simulink model "testrig_quarter_car"  (R2025b)
settings: Solver=ode23t  StartTime=0.0  StopTime=96  MaxStep=0.1  RelTol=1e-3  AbsTol=1e-3  EnableMultiTasking=on
PostLoadFcn:
  | Maneuver = MDatabase.KnC.FSAE_Achilles;
values from neighbouring files (symbols this model uses):
  Vehicle = evalin('base','Vehicle')    [sm_car_knc_plot1toecamber.m]    (also in testrig_quarter_car_results.m = sm_car_vehcfg_setPeopleOnOff(Vehicle,[0 0 0 0 0],'SuspA1'))
undefined symbols (not defined in the file or in its folder): X, Y, Z
libraries: sm_lib x9, nesl_utility x6, fl_lib x6, sm_car_testrig_utilities_lib x5, Damper_Element x1, Linkage_Systems x1, Suspension_Utilities x1
CloseFcn:
  | clear simlog_sm_car_testrig_quarter_car
  | clear logsout_sm_car_testrig_quarter_car
  | evalin('base','Maneuver = MDatabase.Skidpad.FSAE_Achilles;')
Description:
  | Copyright 2020-2024 The MathWorks, Inc.
settings Model: Creator=smiller  LastModifiedBy=andrei
settings SolverCC: AutoScaleAbsTol=off  AlgebraicLoopSolver=TrustRegion
settings DataIOCC: LimitDataPoints=on  MaxDataPoints=10000  ReturnWorkspaceOutputs=off  SignalLoggingName=logsout_sm_car_testrig_quarter_car
settings OptimizationCC: LifeSpan=inf
settings DebuggingCC: UnconnectedInputMsg=warning  UnconnectedOutputMsg=warning  UnconnectedLineMsg=warning  AllowSymbolicDim=off  SFUnexpectedBacktrackingDiag=warning  SFNoUnconditionalDefaultTransitionDiag=warning  SFExecutionAtInitializationDiag=none  ArithmeticOperatorsInVariantConditions=warning
settings ModelReferenceCC: EnableRefExpFcnMdlSchedulingChecks=on
settings SFSimCC: SimUseLocalCustomCode=off  CustomCodeUndefinedFunction=UseInterfaceOnly
settings RTWCC: RTWUseLocalCustomCode=off  GPUComputeCapability=3.5
settings CodeAppCC: StateflowObjectComments=on
settings GRTTargetCC: TargetLangStandard=C89/C90 (ANSI)
settings ConfigComp: CovMetricSettings=dw  CovSaveCumulativeToWorkspaceVar=on  CovSaveSingleToWorkspaceVar=on  CovExternalEMLEnable=off  CovSFcnEnable=off
settings SimscapeCC: SimscapeLogType=all  SimscapeLogSimulationStatistics=on  SimscapeLogName=simlog_sm_car_testrig_quarter_car  SimscapeLogDataHistory=10000.0
settings DiagnosticsConfigSet: SimMechanicsUnconnectedFramePorts=none
settings ExplorerConfigSet: InternalSimMechanicsExplorerSettings="<ExplorerConfiguration><canonicalview>default</canonicalview><AnimationSetting><BasePlaybackSpeed>1.0</BasePlaybackSpeed><PlaybackSpeedFactor>16.0</PlaybackSpeedFactor></AnimationSetting><TilePanel><TileInfo><Tiles Columns=\"1\" Count=\"1\" Rows=\"1\"><Column Weight=\"1\"/><Row Weight=\"1\"/><Tile Height=\"1\" Width=\"1\" X=\"0\" Y=\"0\"/></Tiles></TileInfo><SceneInfo><SceneViewer><BGColor><R>1</R><G>1</G><B>1</B></BGColor><Camera><DoPerspective>off</DoPerspective><Position><X>-1.00754384696483612</X><Y>0.620980322360992432</Y><Z>0.415903732180595842</Z></Position><Center><X>-0.00754384696483612061</X><Y>0.620980322360992432</Y><Z>0.415903732180595842</Z></Center><Up><X>0</X><Y>0</Y><Z>1</Z></Up><ViewLimDist>1</ViewLimDist><YLim>0.446366462798987951</YLim><XLim>0.523904299059845036</XLim></Camera></SceneViewer></SceneInfo></TilePanel><MechEditorPanel><Cameras/><GfxPanelCameraMap/><VideoCreator><PlaybackSpeedRatio>1.0</PlaybackSpeedRatio><FrameRate>30</FrameRate><VideoFormat>Motion JPEG AVI</VideoFormat><FrameSize>auto</FrameSize></VideoCreator></MechEditorPanel></ExplorerConfiguration>"

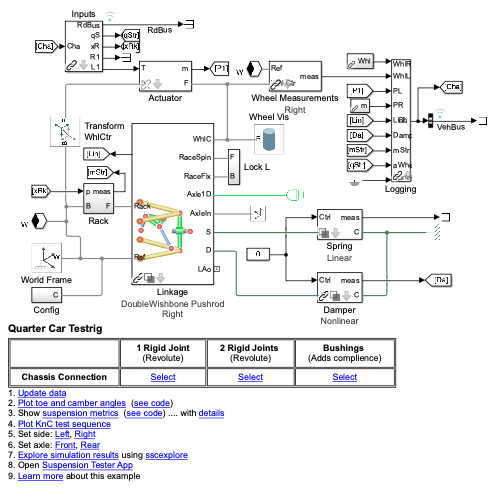
[thumbnail: Simulink's stored preview of the top-level diagram]
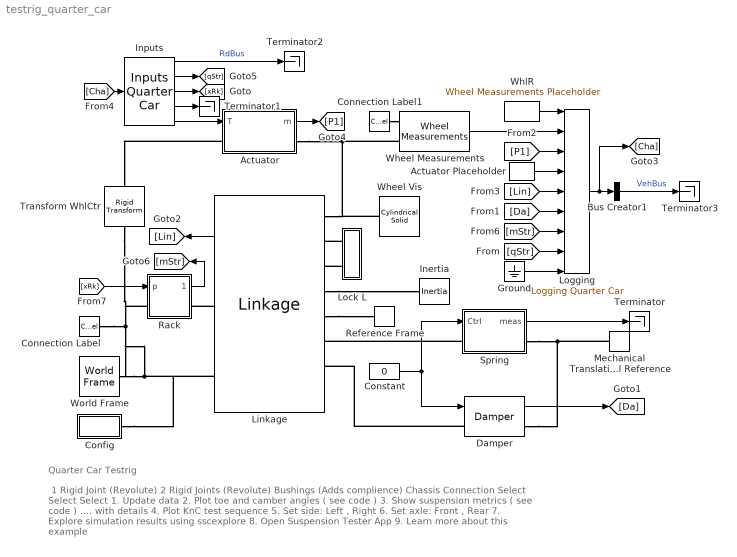
== system testrig_quarter_car ==
  note: Quarter Car Testrig
  note: ​
      | 1 Rigid Joint
      | (Revolute)
      | 2 Rigid Joints
      | (Revolute)
      | Bushings
      | (Adds complience)
      |
      | Chassis Connection
      | Select
      | Select
      | Select
      |
      | 1. Update data
      | 2. Plot toe and camber angles ( see code )
      | 3. Show suspension metrics ( see code ) .... with details
      | 4. Plot KnC test sequence
      | 5. Set side: Left , Right
      | 6. Set axle: Front , Rear
      | 7. Explore simulation results using sscexplore
      | 8. Open Suspension Tester App
      | 9. Learn more about this example
  Actuator : Subsystem  AncestorBlock=sm_car_testrig_utilities_lib/Actuator Quarter Car  mask{veh=Vehicle, xCPOffset=Maneuver.xCPOffset, tir_file=Vehicle.Chassis.Tire.tirFile.Value}
      mask prompts: veh "Vehicle (structure)"; xCPOffset "xOffset from Contact Patch for force test (m)"; tir_file "Tire File"
      mask init:
      | tire_param = simscape.multibody.tirread(eval(tir_file));
      | tire_radius = tire_param.DIMENSION.UNLOADED_RADIUS;
      mask TypeOptions xCPOffset: Actuator/xCPOffset
  Actuator Placeholder : sm_car_testrig_utilities_lib/Actuator Placeholder  SystemSampleTime=-1  VariantActivationTime=update diagram  EmptyChoice=off  PassThrough=off  PassThroughVariantControl=(default)  EmptyChoiceVariantControl=(default)  AllowFlexibleInterface=on  Latency=0  AutoFrameSizeCalculation=off
  Bus Creator1 : BusCreator  Inputs=1
  Config : Subsystem
  Connection Label : ConnectionLabel  Label=W
  Connection Label1 : ConnectionLabel  Label=W
  Constant : Constant  Value=0
  Damper : Damper_Element/Damper  VariantControl=Variant1  LabelModeActiveChoice=Nonlinear  Damper=Vehicle.Chassis.Damper.Axle1  VariantLabel=Vehicle.Chassis.Damper.Axle1.class.Value
      settings: AttributesFormatString=%<ActiveVariant>
  Ground : Ground
  Inertia : fl_lib/Mechanical/Rotational Elements/Inertia  inertia=0.01 kg*m^2  num_ports=foundation.enum.numPorts2.one  w_specify=on  w_priority=None  w=0 rad/s  w_nominal_specify=off  w_nominal_value=1  w_nominal_unit=rad/s  t_specify=off  t_priority=None  t=0 N*m  t_nominal_specify=off  t_nominal_value=1  t_nominal_unit=N*m
  Inputs : sm_car_testrig_utilities_lib/Inputs Quarter Car  popup_steering_input=On
  Linkage : Linkage_Systems/Linkage  VariantControl=Variant1  LabelModeActiveChoice=DoubleWishbone Pushrod  popup_leftRight=Right  Linkage=Vehicle.Chassis.SuspA1.Linkage  InitLinkage=Init.Axle1  VariantLabel=Vehicle.Chassis.SuspA1.Linkage.class.Value
      settings: AttributesFormatString=|
      | %<ActiveVariant>
      | %<popup_leftRight>
  Lock L : Subsystem
  Logging : sm_car_testrig_utilities_lib/Logging Quarter Car
  Mechanical Translational Reference : fl_lib/Mechanical/Translational Elements/Mechanical Translational Reference
  Rack : Subsystem
  Reference Frame : sm_lib/Frames and Transforms/Reference Frame
  Spring : Subsystem  Variant=on  VariantControlMode=label  VariantControl=Variant1  LabelModeActiveChoice=Linear  mask(Variants for Spring){Spring=Vehicle.Chassis.Spring.Axle1, VariantLabel=Vehicle.Chassis.Spring.Axle1.class.Value}
      mask prompts: Spring "Spring Parameters"; VariantLabel "Variant Label"
      mask help: Select option and provide parameters for spring. Option is chosen by string provided in Variant Label. The parameters for the selected option is contained in Spring data structure.
      mask init:
      | curblk = gcb;
      | 
      | % Set variant for this block 
      | set_param(curblk,'LabelModeActiveChoice',VariantLabel);
      settings: AttributesFormatString=%<ActiveVariant>
      mask Display: disp(' ')
  Terminator{,1..3} (4 alike) : Terminator
  Transform WhlCtr : sm_lib/Frames and Transforms/Rigid Transform  RotationMethod=None  FollAlignAxisA=+X  BaseAlignAxisA=+Y  FollAlignAxisB=+Y  BaseAlignAxisB=+Z  RotationStandardAxis=+Z  RotationAngle=0.0  RotationAngleUnits=deg  RotationArbitraryAxis=[0 0 1]  RotationSequenceAxes=FollowerAxes  RotationSequence=XYX  RotationSequenceAngles=[0 0 0]  RotationSequenceAnglesUnits=deg  RotationMatrix=[1 0 0; 0 1 0; 0 0 1]  Quaternion=[1 0 0 0]  TranslationMethod=StandardAxis  TranslationCartesianOffset=[0 0 0]  TranslationCartesianOffsetUnits=m  TranslationStandardAxis=+Z  TranslationStandardOffset=Vehicle.Chassis.SuspA1.Linkage.Upright.sWheelCentre.Value(3)  TranslationStandardOffsetUnits=m  TranslationROffset=0  TranslationROffsetUnits=m  TranslationThetaOffset=0  TranslationThetaOffsetUnits=deg  TranslationZOffset=0  TranslationZOffsetUnits=m
  Wheel Measurements : Suspension_Utilities/Wheel Measurements  popup_leftRight=Right
      settings: AttributesFormatString=%<popup_leftRight>  SourceProductName=SmCar - Suspension Utilites
  Wheel Vis : sm_lib/Body Elements/Cylindrical Solid  CylinderRadius=0.23  CylinderRadiusUnits=m  CylinderLength=0.25  CylinderLengthUnits=m  ExportEntireGeometry=off  InertiaType=CalculateFromGeometry  BasedOnType=Mass  Density=1000  DensityUnits=kg/m^3  Mass=10  MassUnits=kg  CenterOfMass=[0 0 0]  CenterOfMassUnits=m  MomentsOfInertia=[1 1 1]  MomentsOfInertiaUnits=kg*m^2  ProductsOfInertia=[0 0 0]  ProductsOfInertiaUnits=kg*m^2  GraphicType=FromGeometry  MarkerShape=Sphere  MarkerSize=10  GraphicVisPropType=SimpleVisualProperties  GraphicDiffuseColor=[0.5 0.5 0.5]  GraphicOpacity=0.3  GraphicSpecularColor=[0.5 0.5 0.5 1.0]  GraphicAmbientColor=[0.15 0.15 0.15 1.0]  GraphicEmissiveColor=[0.0 0.0 0.0 1.0]  GraphicShininess=75  DoExposeReferenceFrame=on  SerializedFrames=<Frames/>
  WhlR : sm_car_testrig_utilities_lib/Wheel Measurements Placeholder  SystemSampleTime=-1  VariantActivationTime=update diagram  EmptyChoice=off  PassThrough=off  PassThroughVariantControl=(default)  EmptyChoiceVariantControl=(default)  AllowFlexibleInterface=on  Latency=0  AutoFrameSizeCalculation=off
  World Frame : sm_lib/Frames and Transforms/World Frame
  wires:
  Constant/1 -> Spring/1("Ctrl "), Damper/1
  Spring/1(" meas") -> Terminator/1
  Linkage/1 -> [Lin]
  Bus Creator1/1 -> Terminator3/1  "VehBus"
  [xRk] -> Rack/1(p)
  Damper/1 -> [Da]
  Wheel Measurements/1 -> Logging/2
  Inputs/1 -> Terminator2/1  "RdBus"
  Inputs/3 -> [xRk]
  Inputs/4 -> Terminator1/1
  [Cha] -> Inputs/1
  Inputs/2 -> [qStr]
  Logging/1 -> [Cha], Bus Creator1/1
  [qStr] -> Logging/8
  [mStr] -> Logging/7
  [Da] -> Logging/6
  [Lin] -> Logging/5
  [P1] -> Logging/3
  WhlR/1 -> Logging/1
  Ground/1 -> Logging/9
  Actuator Placeholder/1 -> Logging/4
  Rack/1(meas) -> [mStr]
  Inputs/5 -> Actuator/1(T)
  Actuator/1(m) -> [P1]
  connections:
  Wheel Vis/RConn1 -- Linkage/LConn1 -- Actuator/RConn1 -- Wheel Measurements/LConn2
  Mechanical Translational Reference/LConn1 -- Spring/RConn1 -- Damper/RConn1
  World Frame/RConn1 -- Linkage/RConn2 -- Config/RConn1 -- Rack/LConn1 -- Transform WhlCtr/LConn1 -- Connection Label/LConn1
  Spring/LConn1 -- Linkage/LConn6
  Linkage/LConn4 -- Inertia/LConn1
  Linkage/LConn5 -- Reference Frame/RConn1
  Damper/LConn1 -- Linkage/LConn7
  Linkage/RConn1 -- Rack/RConn1
  Lock L/LConn1 -- Linkage/LConn2
  Lock L/LConn2 -- Linkage/LConn3
  Connection Label1/LConn1 -- Wheel Measurements/LConn1
  Actuator/LConn1 -- Transform WhlCtr/RConn1

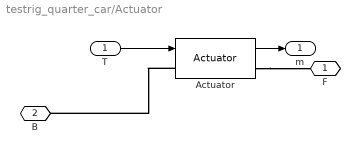
== system testrig_quarter_car/Actuator ==
  T : Inport
  Actuator : sm_car_testrig_utilities_lib/Actuator  tire_rad=tire_radius  xCPOffset=xCPOffset
  F : PMIOPort  Side=Right
  B : PMIOPort  Port=2  Side=Left
  m : Outport
  wires:
  T/1 -> Actuator/1
  Actuator/1 -> m/1
  connections:
  Actuator/RConn1 -- F/RConn1
  Actuator/LConn1 -- B/RConn1

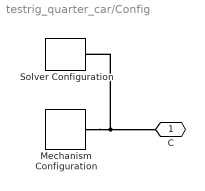
== system testrig_quarter_car/Config ==
  Mechanism Configuration : sm_lib/Utilities/Mechanism Configuration  UniformGravity=Constant  GravityVector=[0 0 -9.80665]  GravityVectorUnits=m/s^2  LinearizationDelta=0.001  JointModeTransitionNonlinearIterations=2
  Solver Configuration : nesl_utility/Solver Configuration  PhysicalDomain=network_engine_domain  SubClassName=solver  LeftPortType=input  RightPortType=generic  Tones=[]  Harmonics=[]  SimulateNoise=off  Profile=off  UseLocalSampling=off  EnableSwitchedLinearOptims=on  FrequencyDomain=off  UseCCode=off  RelTol=0.001  AbsTol=1e-06  MinStep=1e-09  ToWorkspace=off  RevertToSquareIcSolve=off  NumHomotopyIterations=100  PhasorMode=off  PhasorModeNumHarmonics=1  ConsistencySolver=NEWTON_FTOL  IndexReductionMethod=DerivativeReplacement  DoDC=off  ResidualTolerance=1e-09  ConsistencyTolSource=GLOBAL  ConsistencyAbsTol=0.001  ConsistencyRelTol=0.001  ConsistencyTolFactor=0.001  UseLocalSolver=off  LocalSolverChoice=NE_BACKWARD_EULER_ADVANCER  ResolveIndetEquations=on  FunctionEvalNumThread=1  LocalSolverSampleTime=0.001  DoFixedCost=off  MaxNonlinIter=3  MaxModeIter=2  ComputeImpulses=off  ImpulseIterations=2  LinearAlgebra=Sparse  LinearAlgebraNumThread=0  EquationFormulation=NE_TIME_EF  DelaysMemoryBudget=1024  AutomaticFiltering=on  FilteringTimeConstant=0.001  PartitionStorageMethod=AS_NEEDED  PartitionMemoryBudget=1024  PartitionMethod=FAST  MultibodyUseLocalSolver=off  MultibodyLocalSolverChoice=ODE1  MultibodyLocalSolverSampleTime=0.001
  C : PMIOPort  Side=Right
  connections:
  Mechanism Configuration/RConn1 -- Solver Configuration/RConn1 -- C/RConn1

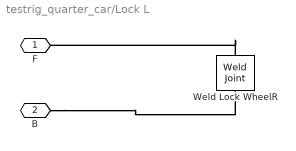
== system testrig_quarter_car/Lock L ==
  Weld Lock WheelR : sm_lib/Joints/Weld Joint  JointMode=Normal  CompositeWrenchDir=FollowerOnBase  CompositeWrenchFrame=BaseFrame  SenseConstraintForce=off  SenseConstraintTorque=off  SenseTotalForce=off  SenseTotalTorque=off
  F : PMIOPort  Side=Left
  B : PMIOPort  Port=2  Side=Left
  connections:
  B/RConn1 -- Weld Lock WheelR/LConn1
  Weld Lock WheelR/RConn1 -- F/RConn1

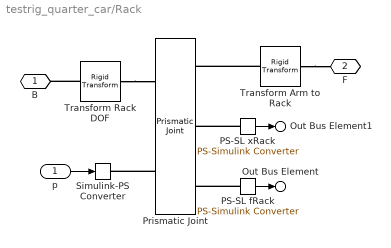
== system testrig_quarter_car/Rack ==
  p : Inport
  PS-SL fRack : nesl_utility/PS-Simulink Converter  PhysicalDomain=network_engine_domain  SubClassName=ps_output  LeftPortType=input  RightPortType=output  PseudoPeriodic=off  Frequencies=[]  VectorFormat=1-D array  Unit=1  AffineConversion=off
  PS-SL xRack : nesl_utility/PS-Simulink Converter  PhysicalDomain=network_engine_domain  SubClassName=ps_output  LeftPortType=input  RightPortType=output  PseudoPeriodic=off  Frequencies=[]  VectorFormat=1-D array  Unit=1  AffineConversion=off
  Prismatic Joint : sm_lib/Joints/Prismatic Joint  JointMode=Normal  CompositeWrenchDir=FollowerOnBase  CompositeWrenchFrame=BaseFrame  SenseConstraintForce=off  SenseConstraintTorque=off  SenseTotalForce=off  SenseTotalTorque=off  PositionTargetSpecify=on  PositionTargetPriority=High  PositionTargetValue=0  PositionTargetValueUnits=m  VelocityTargetSpecify=off  VelocityTargetPriority=High  VelocityTargetValue=0  VelocityTargetValueUnits=m/s  EquilibriumPosition=0  EquilibriumPositionUnits=m  SpringStiffness=0  SpringStiffnessUnits=N/m  DampingCoefficient=0  DampingCoefficientUnits=N/(m/s)  LowerLimitSpecify=off  LowerLimitBound=-1  LowerLimitBoundUnits=m  LowerLimitStiffness=1e6  LowerLimitStiffnessUnits=N/m  LowerLimitDamping=1e3  LowerLimitDampingUnits=N/(m/s)  LowerLimitTransitionRegionWidth=1e-4  LowerLimitTransitionRegionWidthUnits=m  UpperLimitSpecify=off  UpperLimitBound=1  UpperLimitBoundUnits=m  UpperLimitStiffness=1e6  UpperLimitStiffnessUnits=N/m  UpperLimitDamping=1e3  UpperLimitDampingUnits=N/(m/s)  UpperLimitTransitionRegionWidth=1e-4  UpperLimitTransitionRegionWidthUnits=m  TorqueActuationMode=ComputedTorque  MotionActuationMode=InputMotion  SensePosition=on  SenseVelocity=off  SenseAcceleration=off  SenseTorqueForce=on  SenseLowerLimitTorqueForce=off  SenseUpperLimitTorqueForce=off
  Simulink-PS Converter : nesl_utility/Simulink-PS Converter  PhysicalDomain=network_engine_domain  SubClassName=ps_input  LeftPortType=input  RightPortType=output  PseudoPeriodic=off  Frequencies=[]  NoiseDistribution=none  NoiseParameters=[]  Unit=m  AffineConversion=off  FilteringAndDerivatives=filter  SimscapeFilterOrder=2  InputFilterTimeConstant=0.005  UdotUserProvided=0
  Transform Arm to Rack : sm_lib/Frames and Transforms/Rigid Transform  RotationMethod=StandardAxis  FollAlignAxisA=+X  BaseAlignAxisA=+Y  FollAlignAxisB=+Y  BaseAlignAxisB=+Z  RotationStandardAxis=+X  RotationAngle=90  RotationAngleUnits=deg  RotationArbitraryAxis=[0 0 1]  RotationSequenceAxes=FollowerAxes  RotationSequence=XYX  RotationSequenceAngles=[0 0 0]  RotationSequenceAnglesUnits=deg  RotationMatrix=[1 0 0; 0 1 0; 0 0 1]  Quaternion=[1 0 0 0]  TranslationMethod=Cartesian  TranslationCartesianOffset=Vehicle.Chassis.SuspA1.Linkage.TrackRod.sInboard.Value.*[1 0 1]  TranslationCartesianOffsetUnits=m  TranslationStandardAxis=+Z  TranslationStandardOffset=0  TranslationStandardOffsetUnits=m  TranslationROffset=0  TranslationROffsetUnits=m  TranslationThetaOffset=0  TranslationThetaOffsetUnits=deg  TranslationZOffset=0  TranslationZOffsetUnits=m
  Transform Rack DOF : sm_lib/Frames and Transforms/Rigid Transform  RotationMethod=StandardAxis  FollAlignAxisA=+X  BaseAlignAxisA=+Y  FollAlignAxisB=+Y  BaseAlignAxisB=+Z  RotationStandardAxis=+X  RotationAngle=90  RotationAngleUnits=deg  RotationArbitraryAxis=[0 0 1]  RotationSequenceAxes=FollowerAxes  RotationSequence=XYX  RotationSequenceAngles=[0 0 0]  RotationSequenceAnglesUnits=deg  RotationMatrix=[1 0 0; 0 1 0; 0 0 1]  Quaternion=[1 0 0 0]  TranslationMethod=Cartesian  TranslationCartesianOffset=Vehicle.Chassis.SuspA1.Linkage.TrackRod.sInboard.Value.*[1 0 1]  TranslationCartesianOffsetUnits=m  TranslationStandardAxis=+Z  TranslationStandardOffset=0  TranslationStandardOffsetUnits=m  TranslationROffset=0  TranslationROffsetUnits=m  TranslationThetaOffset=0  TranslationThetaOffsetUnits=deg  TranslationZOffset=0  TranslationZOffsetUnits=m
  B : PMIOPort  Side=Left
  F : PMIOPort  Port=2  Side=Right
  Out Bus Element : Outport  VectorParamsAs1DForOutWhenUnconnected=off  PortName=meas  Element=FRack
  Out Bus Element1 : Outport  VectorParamsAs1DForOutWhenUnconnected=off  PortName=meas  Element=xRack
  wires:
  p/1 -> Simulink-PS Converter/1
  PS-SL fRack/1 -> Out Bus Element/1
  PS-SL xRack/1 -> Out Bus Element1/1
  connections:
  Transform Rack DOF/RConn1 -- Prismatic Joint/LConn1
  Prismatic Joint/LConn2 -- Simulink-PS Converter/RConn1
  Transform Arm to Rack/LConn1 -- F/RConn1
  Transform Arm to Rack/RConn1 -- Prismatic Joint/RConn1
  Transform Rack DOF/LConn1 -- B/RConn1
  PS-SL xRack/LConn1 -- Prismatic Joint/RConn2
  PS-SL fRack/LConn1 -- Prismatic Joint/RConn3

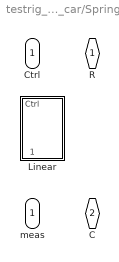
== system testrig_quarter_car/Spring ==
  "Ctrl " : Inport
  Linear : Subsystem  VariantControl=Linear  mask(Linear Spring){spr_def0=Spring.xPreload.Value, spr_k=Spring.K.Value, spr_hp_top=Spring.sTop.Value, spr_hp_bot=Spring.sBottom.Value}
      mask prompts: spr_def0 "Spring Preload (m)"; spr_k "Spring Rate (N/m)"; spr_hp_top "HP Top [xyz] (m)"; spr_hp_bot "HP Bottom [xyz] (m)"
      mask help: Spring with linear stiffness.
      mask init:
      | spr_len0 = norm(spr_hp_top-spr_hp_bot);
  " R" : PMIOPort  Side=Left
  " C" : PMIOPort  Port=2  Side=Right
  " meas" : Outport  VectorParamsAs1DForOutWhenUnconnected=off

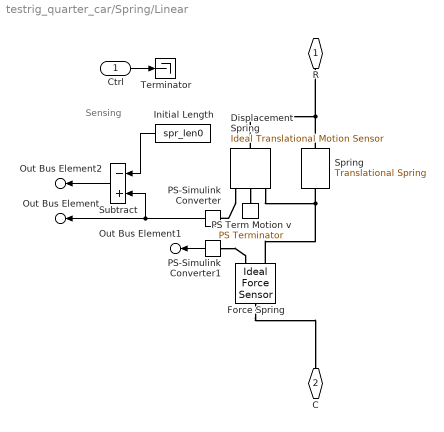
== system testrig_quarter_car/Spring/Linear ==
  note: Sensing
  Ctrl : Inport
  Displacement Spring : fl_lib/Mechanical/Mechanical Sensors/Ideal Translational Motion Sensor  reference=foundation.enum.MeasurementReference.difference  acceleration_port=false  velocity_port=true  position_port=true  offset=spr_len0 m
  Force Spring : fl_lib/Mechanical/Mechanical Sensors/Ideal Force Sensor
  Initial Length : Constant  Value=spr_len0
  PS Term Motion v : fl_lib/Physical Signals/Sinks/PS Terminator
  PS-Simulink Converter : nesl_utility/PS-Simulink Converter  PhysicalDomain=network_engine_domain  SubClassName=ps_output  LeftPortType=input  RightPortType=output  PseudoPeriodic=off  Frequencies=[]  VectorFormat=1-D array  Unit=m  AffineConversion=off
  PS-Simulink Converter1 : nesl_utility/PS-Simulink Converter  PhysicalDomain=network_engine_domain  SubClassName=ps_output  LeftPortType=input  RightPortType=output  PseudoPeriodic=off  Frequencies=[]  VectorFormat=1-D array  Unit=N  AffineConversion=off
  Spring : fl_lib/Mechanical/Translational Elements/Translational Spring  spr_rate=spr_k N/m  v_specify=off  v_priority=None  v=0 m/s  v_nominal_specify=off  v_nominal_value=1  v_nominal_unit=m/s  f_specify=off  f_priority=None  f=0 N  f_nominal_specify=off  f_nominal_value=1  f_nominal_unit=N  x_specify=on  x_priority=High  x=-spr_def0 m  x_nominal_specify=off  x_nominal_value=1  x_nominal_unit=m
  Subtract : Sum  Inputs=-+
  Terminator : Terminator
  R : PMIOPort  Side=Left
  C : PMIOPort  Port=2  Side=Right
  Out Bus Element : Outport  VectorParamsAs1DForOutWhenUnconnected=off  PortName=meas  Element=xSpring
  Out Bus Element1 : Outport  VectorParamsAs1DForOutWhenUnconnected=off  PortName=meas  Element=FSpring
  Out Bus Element2 : Outport  VectorParamsAs1DForOutWhenUnconnected=off  PortName=meas  Element=DeltaxSpring
  wires:
  PS-Simulink Converter/1 -> Out Bus Element/1, Subtract/2
  Ctrl/1 -> Terminator/1
  PS-Simulink Converter1/1 -> Out Bus Element1/1
  Initial Length/1 -> Subtract/1
  Subtract/1 -> Out Bus Element2/1
  connections:
  Displacement Spring/RConn3 -- PS-Simulink Converter/LConn1
  Displacement Spring/RConn2 -- PS Term Motion v/LConn1
  PS-Simulink Converter1/LConn1 -- Force Spring/RConn2
  Force Spring/LConn1 -- C/RConn1
  Displacement Spring/RConn1 -- Force Spring/RConn1 -- Spring/RConn1
  Displacement Spring/LConn1 -- R/RConn1 -- Spring/LConn1
